simulink model "BEV_Thermal_Management"  (R2025a)
settings: Solver=ode23t  StartTime=0  StopTime=765  MaxStep=5  RelTol=1e-3  AbsTol=1e-3
model workspace: external: MATLAB File BEV_Thermal_Management_param.m (data not in the file)
undefined symbols (not defined in the file): Battery, bulb, cabin_doors_conductivity, cabin_duct_area, cabin_glass_conductivity, cabin_roof_conductivity, cabin_T_init, chiller_area_primary, chiller_N_baffles, chiller_N_tubes, chiller_tube_D, chiller_tube_L, chiller_wall_conductivity, chiller_wall_thickness, compressor_rpm_LUT, condenser_air_area_flow, condenser_air_area_primary, condenser_W, condenser_wall_conductivity, condenser_wall_thickness, coolant_channel_D, coolant_pipe_area, coolant_pipe_D, coolant_T_init, coolant_tank_area, coolant_tank_volume, coolant_valve_D_ratio_max, coolant_valve_D_ratio_min, coolant_valve_displacement, coolant_valve_S_max, cycle, DCDC, Edrive, evaporator_air_area_flow, evaporator_air_area_primary, evaporator_W, evaporator_wall_conductivity, evaporator_wall_thickness, heater_max_power, ModuleType1, outlet, ptc_max_power, pump_speed_max, radiationReflectionShields, radiator_air_area_flow, radiator_air_area_primary, radiator_W, radiator_wall_conductivity, radiator_wall_thickness, refrigerant_alpha_init, refrigerant_pipe_D, transRatio
libraries: fl_lib x264, nesl_utility x91, SimscapeFluids_lib x22, sdl_lib x13, ee_lib x9, nesl_utility_internal x4, slpidlib x3, BatteryProtection x3, batt_lib x2, BatteryCurrentManagement x1, autolibsharedcommon x1, simulink x1
(part 5 of 9)

== system BEV_Thermal_Management/Parallel-Serial Mode Valve ==
  note: Parallel mode flow path: A-D and C-B
      |
      | Serial mode flow path: A-B and C-D
  4-Way Valve : SimscapeFluids_lib/Thermal Liquid/Valves & Orifices/Directional Control Valves/4-Way 3-Position Directional Valve (TL)  open_orifices_pos=fluids.thermal_liquid.valves.directional_control_valves.enum.OpenOrifices4WayPosNeg.PA_BT  open_orifices_neu=fluids.thermal_liquid.valves.directional_control_valves.enum.OpenOrifices4WayNeu.all_closed  open_orifices_neg=fluids.thermal_liquid.valves.directional_control_valves.enum.OpenOrifices4WayPosNeg.PB_AT  neutral_assert_action=simscape.enum.assert.action.none  area_spec=fluids.thermal_liquid.valves.directional_control_valves.enum.area_spec.identical  valve_spec=fluids.thermal_liquid.valves.enum.orifice_spec.linear  del_S_max=coolant_valve_displacement m  area_max=pi * (coolant_valve_D_ratio_max*coolant_pipe_D)^2 / 4 m^2  del_S_TLU=[0 0.002 0.004 0.007 0.017] m  valve_area_TLU=[1e-09, 2.0352e-07, 4.0736e-05, .00011438, .00034356] m^2  del_S_flow_TLU=[0 0.002 0.004 0.007 0.017] m  p_diff_TLU=[-.1, .3, .5, .7] MPa  vol_flow_TLU=[-1e-08, 2.2e-08, 2.8e-08, 3.4e-08; -9e-06, .00015, .0002, .00024; -.00036, .00063, .00081, .00096; -.00054, .00094, .0012, .0014; -.00091, .0016, .002, .0024] m^3/s  mdot_TLU=[-1e-05, 1.7e-05, 2e-05, 2.6e-05; -.002, .0035, .0045, .0053; -.4, .7, .9, 1.06; -1.13, 1.96, 2.5, 3; -3.45, 6, 7.7, 9.13] kg/s  p_diff_TLU_const=[-.1, .3, .5, .7] MPa  vol_flow_TLU_const=[-.0009, .0016, .002, .0024] m^3/s  mdot_TLU_const=[-.9, 1.6, 2, 2.4] kg/s  area_const=1e-4 m^2  T_ref_in=293.15 K  p_ref_in=0.101325 MPa  area_leak=pi * (coolant_valve_D_ratio_min*coolant_pipe_D)^2 / 4 m^2  area=coolant_pipe_area m^2  Cd=0.7  Re_c=12  smoothing_factor=0.01  pressure_recovery=simscape.enum.onoff.on  S_max_PA=coolant_valve_S_max m  del_S_max_PA=coolant_valve_displacement-(coolant_valve_displacement)*(pi * (coolant_valve_D_ratio_min*coolant_pipe_D)^2 / 4)/(pi * (coolant_valve_D_ratio_max*coolant_pipe_D)^2 / 4) m  area_max_PA=pi * (coolant_valve_D_ratio_max*coolant_pipe_D)^2 / 4 m^2  del_S_TLU_PA=[0 0.002 0.004 0.007 0.017] m  valve_area_TLU_PA=[1e-09, 2.0352e-07, 4.0736e-05, .00011438, .00034356] m^2  del_S_flow_TLU_PA=[0 0.002 0.004 0.007 0.017] m  p_diff_TLU_PA=[-.1, .3, .5, .7] MPa  vol_flow_TLU_PA=[-1e-08, 2.2e-08, 2.8e-08, 3.4e-08; -9e-06, .00015, .0002, .00024; -.00036, .00063, .00081, .00096; -.00054, .00094, .0012, .0014; -.00091, .0016, .002, .0024] m^3/s  mdot_TLU_PA=[-1e-05, 1.7e-05, 2e-05, 2.6e-05; -.002, .0035, .0045, .0053; -.4, .7, .9, 1.06; -1.13, 1.96, 2.5, 3; -3.45, 6, 7.7, 9.13] kg/s  area_const_PA=1e-4 m^2  p_diff_TLU_const_PA=[-.1, .3, .5, .7] MPa  vol_flow_TLU_const_PA=[-.0009, .0016, .002, .0024] m^3/s  mdot_TLU_const_PA=[-.9, 1.6, 2, 2.4] kg/s  S_max_PB=-coolant_valve_S_max m  del_S_max_PB=coolant_valve_displacement-(coolant_valve_displacement)*(pi * (coolant_valve_D_ratio_min*coolant_pipe_D)^2 / 4)/(pi * (coolant_valve_D_ratio_max*coolant_pipe_D)^2 / 4) m  area_max_PB=pi * (coolant_valve_D_ratio_max*coolant_pipe_D)^2 / 4 m^2  del_S_TLU_PB=[0 0.002 0.004 0.007 0.017] m  valve_area_TLU_PB=[1e-09, 2.0352e-07, 4.0736e-05, .00011438, .00034356] m^2  del_S_flow_TLU_PB=[0 0.002 0.004 0.007 0.017] m  p_diff_TLU_PB=[-.1, .3, .5, .7] MPa  vol_flow_TLU_PB=[-1e-08, 2.2e-08, 2.8e-08, 3.4e-08; -9e-06, .00015, .0002, .00024; -.00036, .00063, .00081, .00096; -.00054, .00094, .0012, .0014; -.00091, .0016, .002, .0024] m^3/s  mdot_TLU_PB=[-1e-05, 1.7e-05, 2e-05, 2.6e-05; -.002, .0035, .0045, .0053; -.4, .7, .9, 1.06; -1.13, 1.96, 2.5, 3; -3.45, 6, 7.7, 9.13] kg/s  area_const_PB=1e-4 m^2  p_diff_TLU_const_PB=[-.1, .3, .5, .7] MPa  vol_flow_TLU_const_PB=[-.0009, .0016, .002, .0024] m^3/s  mdot_TLU_const_PB=[-.9, 1.6, 2, 2.4] kg/s  S_max_AB=7.5e-3 m  del_S_max_AB=0.005 m  area_max_AB=1e-4 m^2  del_S_TLU_AB=[0, .00125, .0025, .00375, .005] m  valve_area_TLU_AB=[1e-10, 1e-05, 4e-05, 6e-05, .0001] m^2  del_S_flow_TLU_AB=[0, .00125, .0025, .00375, .005] m  p_diff_TLU_AB=[-.1, .3, .5, .7] MPa  vol_flow_TLU_AB=[-1e-08, 2.2e-08, 2.8e-08, 3.4e-08; -9e-06, .00015, .0002, .00024; -.00036, .00063, .00081, .00096; -.00054, .00094, .0012, .0014; -.00091, .0016, .002, .0024] m^3/s  mdot_TLU_AB=[1.7e-05, 2e-05, 2.6e-05; .0035, .0045, .0053; .7, .9, 1.06; 1.96, 2.5, 3; 6, 7.7, 9.13] kg/s  area_const_AB=1e-4 m^2  p_diff_TLU_const_AB=[-.1, .3, .5, .7] MPa  vol_flow_TLU_const_AB=[-.0009, .0016, .002, .0024] m^3/s  mdot_TLU_const_AB=[-.9, 1.6, 2, 2.4] kg/s  S_max_AT=-coolant_valve_S_max m  del_S_max_AT=coolant_valve_displacement-(coolant_valve_displacement)*(pi * (coolant_valve_D_ratio_min*coolant_pipe_D)^2 / 4)/(pi * (coolant_valve_D_ratio_max*coolant_pipe_D)^2 / 4) m  area_max_AT=pi * (coolant_valve_D_ratio_max*coolant_pipe_D)^2 / 4 m^2  del_S_TLU_AT=[0 0.002 0.004 0.007 0.017] m  valve_area_TLU_AT=[1e-09, 2.0352e-07, 4.0736e-05, .00011438, .00034356] m^2  del_S_flow_TLU_AT=[0 0.002 0.004 0.007 0.017] m  p_diff_TLU_AT=[-.1, .3, .5, .7] MPa  vol_flow_TLU_AT=[-1e-08, 2.2e-08, 2.8e-08, 3.4e-08; -9e-06, .00015, .0002, .00024; -.00036, .00063, .00081, .00096; -.00054, .00094, .0012, .0014; -.00091, .0016, .002, .0024] m^3/s  mdot_TLU_AT=[-1e-05, 1.7e-05, 2e-05, 2.6e-05; -.002, .0035, .0045, .0053; -.4, .7, .9, 1.06; -1.13, 1.96, 2.5, 3; -3.45, 6, 7.7, 9.13] kg/s  area_const_AT=1e-4 m^2  p_diff_TLU_const_AT=[-.1, .3, .5, .7] MPa  vol_flow_TLU_const_AT=[-.0009, .0016, .002, .0024] m^3/s  mdot_TLU_const_AT=[-.9, 1.6, 2, 2.4] kg/s  S_max_BT=coolant_valve_S_max m  del_S_max_BT=coolant_valve_displacement-(coolant_valve_displacement)*(pi * (coolant_valve_D_ratio_min*coolant_pipe_D)^2 / 4)/(pi * (coolant_valve_D_ratio_max*coolant_pipe_D)^2 / 4) m  area_max_BT=pi * (coolant_valve_D_ratio_max*coolant_pipe_D)^2 / 4 m^2  del_S_TLU_BT=[0 0.002 0.004 0.007 0.017] m  valve_area_TLU_BT=[1e-09, 2.0352e-07, 4.0736e-05, .00011438, .00034356] m^2  del_S_flow_TLU_BT=[0 0.002 0.004 0.007 0.017] m  p_diff_TLU_BT=[-.1, .3, .5, .7] MPa  vol_flow_TLU_BT=[-1e-08, 2.2e-08, 2.8e-08, 3.4e-08; -9e-06, .00015, .0002, .00024; -.00036, .00063, .00081, .00096; -.00054, .00094, .0012, .0014; -.00091, .0016, .002, .0024] m^3/s  mdot_TLU_BT=[-1e-05, 1.7e-05, 2e-05, 2.6e-05; -.002, .0035, .0045, .0053; -.4, .7, .9, 1.06; -1.13, 1.96, 2.5, 3; -3.45, 6, 7.7, 9.13] kg/s  area_const_BT=1e-4 m^2  p_diff_TLU_const_BT=[-.1, .3, .5, .7] MPa  vol_flow_TLU_const_BT=[-.0009, .0016, .002, .0024] m^3/s  mdot_TLU_const_BT=[-.9, 1.6, 2, 2.4] kg/s  S_max_PT=0 m  del_S_max_PT=0.005 m  area_max_PT=1e-4 m^2  del_S_TLU_PT=[0, .00125, .0025, .00375, .005] m  valve_area_TLU_PT=[1e-10, 1e-05, 4e-05, 6e-05, .0001] m^2  del_S_flow_TLU_PT=[0, .00125, .0025, .00375, .005] m  p_diff_TLU_PT=[-.1, .3, .5, .7] MPa  vol_flow_TLU_PT=[-1e-08, 2.2e-08, 2.8e-08, 3.4e-08; -9e-06, .00015, .0002, .00024; -.00036, .00063, .00081, .00096; -.00054, .00094, .0012, .0014; -.00091, .0016, .002, .0024] m^3/s  mdot_TLU_PT=[1.7e-05, 2e-05, 2.6e-05; .0035, .0045, .0053; .7, .9, 1.06; 1.96, 2.5, 3; 6, 7.7, 9.13] kg/s
      settings: InternalSimscapePortConfiguration="{\"Bottom\":[],\"Left\":[{\"id\":\"A\",\"label\":\"A\",\"type\":\"foundation.thermal_liquid.thermal_liquid\"},{\"id\":\"B\",\"label\":\"B\",\"type\":\"foundation.thermal_liquid.thermal_liquid\"}],\"Right\":[{\"id\":\"S\",\"label\":\"S\",\"type\":\"input\"},{\"id\":\"P\",\"label\":\"P\",\"type\":\"foundation.thermal_liquid.thermal_liquid\"},{\"id\":\"T\",\"label\":\"T\",\"type\":\"foundation.thermal_liquid.thermal_liquid\"}],\"Top\":[]}"
  Battery Coolant Tank : SimscapeFluids_lib/Thermal Liquid/Tanks & Accumulators/Tank (G-TL)  num_inlet=2  volume_total=coolant_tank_volume l  volume_spec=1  tank_area=coolant_tank_area m^2  level_TLU=[0, 3, 5] m  volume_TLU=[0, 4, 6] m^3  inlet_areas_A1B1=[.01, .01] m^2  inlet_height_A2=0.1 m  inlet_area_A2=0.01 m^2  inlet_heights_A2B2=[0, 0] m  inlet_areas_A2B2=[1 1] * coolant_pipe_area m^2  inlet_heights_A2B2C2=[.1, .1, .1] m  inlet_areas_A2B2C2=[.01, .01, .01] m^2  inlet_heights_A2B2C2D2=0.1 * ones(1, 4) m  inlet_areas_A2B2C2D2=0.01 * ones(1, 4) m^2  inlet_heights_A2B2C2D2E2=0.1 * ones(1, 5) m  inlet_areas_A2B2C2D2E2=0.01 * ones(1, 5) m^2  inlet_heights_A2B2C2D2E2F2=0.1 * ones(1, 6) m  inlet_areas_A2B2C2D2E2F2=0.01 * ones(1, 6) m^2  capacity_check=0  max_liquid_capacity=coolant_tank_volume l  g=0 m/s^2  level_specify=on  level_priority=None  level=5 m  level_nominal_specify=off  level_nominal_value=1  level_nominal_unit=m  volume_liquid_specify=on  volume_liquid_priority=High  volume_liquid=0.25 * coolant_tank_volume l  volume_liquid_nominal_specify=off  volume_liquid_nominal_value=1  volume_liquid_nominal_unit=m^3  mass_liquid_specify=off  mass_liquid_priority=None  mass_liquid=5e+3 kg  mass_liquid_nominal_specify=off  mass_liquid_nominal_value=1  mass_liquid_nominal_unit=kg  T_liquid_specify=on  T_liquid_priority=High  T_liquid=coolant_T_init K  T_liquid_nominal_specify=off  T_liquid_nominal_value=1  T_liquid_nominal_unit=K  p_gas_specify=on  p_gas_priority=High  p_gas=coolant_p_init MPa  p_gas_nominal_specify=off  p_gas_nominal_value=1  p_gas_nominal_unit=MPa  T_gas_specify=on  T_gas_priority=High  T_gas=coolant_T_init K  T_gas_nominal_specify=off  T_gas_nominal_value=1  T_gas_nominal_unit=K  rho_gas_specify=off  rho_gas_priority=None  rho_gas=1.2 kg/m^3  rho_gas_nominal_specify=off  rho_gas_nominal_value=1  rho_gas_nominal_unit=kg/m^3
      settings: InternalSimscapePortConfiguration="{\"Bottom\":[],\"Left\":[{\"id\":\"A1\",\"label\":\"A1\",\"type\":\"foundation.gas.gas\"},{\"id\":\"B1\",\"label\":\"B1\",\"type\":\"foundation.gas.gas\"},{\"id\":\"A2\",\"label\":\"A2\",\"type\":\"foundation.thermal_liquid.thermal_liquid\"},{\"id\":\"B2\",\"label\":\"B2\",\"type\":\"foundation.thermal_liquid.thermal_liquid\"}],\"Right\":[{\"id\":\"H1\",\"label\":\"H1\",\"type\":\"foundation.thermal.thermal\"},{\"id\":\"H2\",\"label\":\"H2\",\"type\":\"foundation.thermal.thermal\"}],\"Top\":[{\"id\":\"V_out\",\"label\":\"V\",\"type\":\"output\"},{\"id\":\"L_out\",\"label\":\"L\",\"type\":\"output\"}]}"
  Battery Coolant Tank Heat Transfer : Subsystem
  Bias : Bias  Bias=-1  SaturateOnIntegerOverflow=off
  Cap (G){,1..3} (4 alike) : fl_lib/Gas/Elements/Cap (G)  p_specify=off  p_priority=None  p=0.101325 MPa  p_nominal_specify=off  p_nominal_value=1  p_nominal_unit=MPa  T_specify=off  T_priority=None  T=293.15 K  T_nominal_specify=off  T_nominal_value=1  T_nominal_unit=K
  Coolant Properties : SimscapeFluids_lib/Thermal Liquid/Utilities/Thermal Liquid Properties (TL)  fluid_list=fluids.thermal_liquid.utilities.enum.thermal_liquid_fluid_list.ethylene_glycol  concentration_param_EG=fluids.thermal_liquid.utilities.enum.thermal_liquid_concentration.volume_fraction  concentration_param_PG=fluids.thermal_liquid.utilities.enum.thermal_liquid_concentration.volume_fraction  c_mass_SW=3.5e-3  c_mass_EG=0.1  c_mass_PG=0.1  c_mass_GL=0.1  c_vol_EG=0.4  c_vol_PG=0.1  beta_const_EG=2.1791 GPa  beta_const_PG=2.1791 GPa  beta_const_GL=2.1791 GPa  p_min_EG=0.01 MPa  p_min_PG=0.01 MPa  p_min_GL=0.01 MPa  p_max_EG=50 MPa  p_max_PG=50 MPa  p_max_GL=50 MPa  p_atm=0.101325 MPa  properties_range_check=simscape.enum.assert.action.error
  Coolant Properties2 : SimscapeFluids_lib/Thermal Liquid/Utilities/Thermal Liquid Properties (TL)  Commented=on  fluid_list=fluids.thermal_liquid.utilities.enum.thermal_liquid_fluid_list.ethylene_glycol  concentration_param_EG=fluids.thermal_liquid.utilities.enum.thermal_liquid_concentration.volume_fraction  concentration_param_PG=fluids.thermal_liquid.utilities.enum.thermal_liquid_concentration.volume_fraction  c_mass_SW=3.5e-3  c_mass_EG=0.1  c_mass_PG=0.1  c_mass_GL=0.1  c_vol_EG=0.5  c_vol_PG=0.1  beta_const_EG=2.1791 GPa  beta_const_PG=2.1791 GPa  beta_const_GL=2.1791 GPa  p_min_EG=0.01 MPa  p_min_PG=0.01 MPa  p_min_GL=0.01 MPa  p_max_EG=50 MPa  p_max_PG=50 MPa  p_max_GL=50 MPa  p_atm=0.101325 MPa  properties_range_check=simscape.enum.assert.action.error
  Gain : Gain  Gain=2
  Max Valve Displacement [m] : Gain  Gain=coolant_valve_displacement
  Motor Coolant Tank : SimscapeFluids_lib/Thermal Liquid/Tanks & Accumulators/Tank (G-TL)  num_inlet=2  volume_total=coolant_tank_volume l  volume_spec=1  tank_area=coolant_tank_area m^2  level_TLU=[0, 3, 5] m  volume_TLU=[0, 4, 6] m^3  inlet_areas_A1B1=[.01, .01] m^2  inlet_height_A2=0.1 m  inlet_area_A2=0.01 m^2  inlet_heights_A2B2=[0, 0] m  inlet_areas_A2B2=[1 1] * coolant_pipe_area m^2  inlet_heights_A2B2C2=[.1, .1, .1] m  inlet_areas_A2B2C2=[.01, .01, .01] m^2  inlet_heights_A2B2C2D2=0.1 * ones(1, 4) m  inlet_areas_A2B2C2D2=0.01 * ones(1, 4) m^2  inlet_heights_A2B2C2D2E2=0.1 * ones(1, 5) m  inlet_areas_A2B2C2D2E2=0.01 * ones(1, 5) m^2  inlet_heights_A2B2C2D2E2F2=0.1 * ones(1, 6) m  inlet_areas_A2B2C2D2E2F2=0.01 * ones(1, 6) m^2  capacity_check=0  max_liquid_capacity=coolant_tank_volume l  g=0 m/s^2  level_specify=on  level_priority=None  level=5 m  level_nominal_specify=off  level_nominal_value=1  level_nominal_unit=m  volume_liquid_specify=on  volume_liquid_priority=High  volume_liquid=0.25 * coolant_tank_volume l  volume_liquid_nominal_specify=off  volume_liquid_nominal_value=1  volume_liquid_nominal_unit=m^3  mass_liquid_specify=off  mass_liquid_priority=None  mass_liquid=5e+3 kg  mass_liquid_nominal_specify=off  mass_liquid_nominal_value=1  mass_liquid_nominal_unit=kg  T_liquid_specify=on  T_liquid_priority=High  T_liquid=coolant_T_init K  T_liquid_nominal_specify=off  T_liquid_nominal_value=1  T_liquid_nominal_unit=K  p_gas_specify=on  p_gas_priority=High  p_gas=coolant_p_init MPa  p_gas_nominal_specify=off  p_gas_nominal_value=1  p_gas_nominal_unit=MPa  T_gas_specify=on  T_gas_priority=High  T_gas=coolant_T_init K  T_gas_nominal_specify=off  T_gas_nominal_value=1  T_gas_nominal_unit=K  rho_gas_specify=off  rho_gas_priority=None  rho_gas=1.2 kg/m^3  rho_gas_nominal_specify=off  rho_gas_nominal_value=1  rho_gas_nominal_unit=kg/m^3
      settings: InternalSimscapePortConfiguration="{\"Bottom\":[],\"Left\":[{\"id\":\"A1\",\"label\":\"A1\",\"type\":\"foundation.gas.gas\"},{\"id\":\"B1\",\"label\":\"B1\",\"type\":\"foundation.gas.gas\"},{\"id\":\"A2\",\"label\":\"A2\",\"type\":\"foundation.thermal_liquid.thermal_liquid\"},{\"id\":\"B2\",\"label\":\"B2\",\"type\":\"foundation.thermal_liquid.thermal_liquid\"}],\"Right\":[{\"id\":\"H1\",\"label\":\"H1\",\"type\":\"foundation.thermal.thermal\"},{\"id\":\"H2\",\"label\":\"H2\",\"type\":\"foundation.thermal.thermal\"}],\"Top\":[{\"id\":\"V_out\",\"label\":\"V\",\"type\":\"output\"},{\"id\":\"L_out\",\"label\":\"L\",\"type\":\"output\"}]}"
  Motor Coolant Tank Heat Transfer : Subsystem
  Simulink-PS Converter : nesl_utility/Simulink-PS Converter  PhysicalDomain=network_engine_domain  SubClassName=ps_input  LeftPortType=input  RightPortType=output  PseudoPeriodic=off  Frequencies=[]  NoiseDistribution=none  NoiseParameters=[]  Unit=m  AffineConversion=off  FilteringAndDerivatives=provide  SimscapeFilterOrder=1  InputFilterTimeConstant=0.001  UdotUserProvided=0
  Transfer Fcn : TransferFcn  Denominator=[1 1]
  D : PMIOPort  Side=Left
  A : PMIOPort  Port=2  Side=Left
  B : PMIOPort  Port=3  Side=Right
  C : PMIOPort  Port=4  Side=Right
  wires:
  [cmd_parallel_serial] -> Transfer Fcn/1
  Gain/1 -> Bias/1
  Bias/1 -> Max Valve Displacement [m]/1
  Max Valve Displacement [m]/1 -> Simulink-PS Converter/1
  Transfer Fcn/1 -> Gain/1
  connections:
  4-Way Valve/RConn3 -- Coolant Properties/RConn1 -- Coolant Properties2/RConn1 -- C/RConn1
  4-Way Valve/RConn1 -- Simulink-PS Converter/RConn1
  4-Way Valve/LConn2 -- Motor Coolant Tank/LConn3
  Cap (G)1/LConn1 -- Motor Coolant Tank/LConn2
  Cap (G)/LConn1 -- Motor Coolant Tank/LConn1
  Motor Coolant Tank Heat Transfer/RConn1 -- Motor Coolant Tank/RConn1
  Motor Coolant Tank Heat Transfer/RConn2 -- Motor Coolant Tank/RConn2
  D/RConn1 -- Motor Coolant Tank/LConn4
  Cap (G)2/LConn1 -- Battery Coolant Tank/LConn1
  Cap (G)3/LConn1 -- Battery Coolant Tank/LConn2
  B/RConn1 -- Battery Coolant Tank/LConn4
  4-Way Valve/LConn1 -- Battery Coolant Tank/LConn3
  Battery Coolant Tank Heat Transfer/LConn1 -- Battery Coolant Tank/RConn1
  Battery Coolant Tank Heat Transfer/LConn2 -- Battery Coolant Tank/RConn2
  4-Way Valve/RConn2 -- A/RConn1

== system BEV_Thermal_Management/Radiator ==
  note: The radiator dissipates the heat to the ambient air. This is achieved by air flowing through the radiator. The airflow depends from the fan placed close to the radiator and the vehicle speed
  Air Intake : fl_lib/Moist Air/Elements/Flow Resistance (MA)  delta_p_nominal=5e-4 MPa  mdot_nominal=1 kg/s  rho_nominal=1.2 kg/m^3  area=cabin_duct_area m^2  laminar_fraction=1e-3
  Environment Air : fl_lib/Moist Air/Elements/Reservoir (MA)  pressure_input=true  pressure_spec=foundation.enum.pressure_spec.atmospheric  reservoir_pressure=0.101325 MPa  temperature_input=true  temperature_spec=foundation.enum.temperature_spec.atmospheric  reservoir_temperature=293.15 K  humidity_input=true  humidity_spec=foundation.enum.HumiditySpec.RelativeHumidity  reservoir_RH=0.5  reservoir_x_w=0.01  reservoir_y_w=0.01  reservoir_HR=0.01  reservoir_Tw=287 K  trace_gas_input=true  trace_gas_spec=foundation.enum.trace_gas_spec.mole_fraction  reservoir_x_g=0.001  reservoir_y_g=0.001  water_droplets_input=false  reservoir_r_d=0  RH_ws=1  area_A=cabin_duct_area m^2  input_error_spec=foundation.enum.input_range_error.warn
      settings: InternalSimscapePortConfiguration="{\"Bottom\":[],\"Left\":[{\"id\":\"A\",\"label\":\"A\",\"type\":\"foundation.moist_air.moist_air\"}],\"Right\":[{\"id\":\"T\",\"label\":\"T\",\"type\":\"input\"},{\"id\":\"P\",\"label\":\"P\",\"type\":\"input\"},{\"id\":\"W\",\"label\":\"W\",\"type\":\"input\"},{\"id\":\"G\",\"label\":\"G\",\"type\":\"input\"}],\"Top\":[]}"
  Moist Air Properties : fl_lib/Moist Air/Utilities/Moist Air Properties (MA)  R_a=287.047 J/kg/K  T_TLU=[-56.55, -50 : 10 : -10, -5 : 1 : 5, 10 : 10 : 350]' degC  h_a_TLU=[342.416126230579; 349.005511058471; 359.063577249119; 369.119948684177; 379.175469465129; 389.230944678417; 394.258910928084; 395.264534937366; 396.27017101329; 397.275819932805; 398.281482472874; 399.287159410541; 400.292851523015; 401.298559587728; 402.304284382408; 403.310026685143; 404.315787274435; 409.34489180313; 419.404921755863; 429.468036401264; 439.535033154839; 449.606720928652; 459.683919949603; 469.767460521911; 479.858181001348; 489.956925196484; 500.064539372946; 510.181869006204; 520.309755403634; 530.449032296018; 540.60052248087; 550.765034584465; 560.943359995745; 571.136270013102; 581.344513234296; 591.568813210327; 601.809866375885; 612.068340261954; 622.344871990218; 632.640067043998; 642.95449830646; 653.288705353699; 663.643193987949; 674.018435994423; 684.414869104228; 694.832897145098; 705.272890361557; 715.735185886199; 726.220088344236; 736.727870574087; 747.258774447567; 757.813011774199] kJ/kg  mu_a_TLU=[14.2568883320012; 14.6140127728333; 15.1517277055779; 15.6806860159119; 16.2012351072083; 16.7137043125028; 16.9670071730589; 17.017438062815; 17.0677930842452; 17.1180725309876; 17.1682766951315; 17.2184058672268; 17.2684603362935; 17.3184403898301; 17.3683463138234; 17.4181783927569; 17.4679369096204; 17.7156358640698; 18.2056751785154; 18.68879035749; 19.1652344664982; 19.6352478927873; 20.099059103658; 20.5568853601578; 21.0089333871663; 21.4554000014051; 21.8964726992323; 22.3323302062775; 22.7631429910631; 23.1890737447833; 23.6102778293792; 24.0269036959922; 24.4390932757886; 24.8469823450548; 25.2507008663546; 25.6503733074314; 26.0461189394339; 26.4380521159325; 26.8262825340948; 27.2109154792923; 27.5920520543128; 27.969789394274; 28.3442208682439; 28.7154362685068; 29.0835219883356; 29.4485611890712; 29.8106339572472; 30.1698174524429; 30.5261860464955; 30.8798114546565; 31.2307628592324; 31.5791070262086] s*uPa  k_a_TLU=[19.8808489374933; 20.4162454629695; 21.2248743590758; 22.0232452890903; 22.8117314495857; 23.5906913619588; 23.9767075412237; 24.053639990175; 24.1304826682191; 24.2072359051629; 24.2839000294007; 24.3604753679152; 24.4369622462801; 24.5133609886625; 24.5896719178249; 24.6658953551279; 24.7420316205333; 25.1214164701832; 25.8738283029331; 26.6180150229276; 27.3542674377332; 28.0828634735341; 28.8040686837224; 29.5181367785657; 30.2253101618423; 30.9258204644224; 31.6198890677835; 32.3077276126633; 32.9895384896798; 33.6655153099498; 34.33584335461; 35.0007000027879; 35.6602551380254; 36.3146715334901; 36.9641052165342; 37.6087058133173; 38.248616874307; 38.8839761815308; 39.5149160384798; 40.1415635435708; 40.7640408480637; 41.3824653993118; 41.9969501701893; 42.6076038755117; 43.2145311762238; 43.8178328720941; 44.4176060836121; 45.013944423749; 45.6069381602018; 46.1966743687041; 46.783237077953; 47.3667074066625] mW/m/K  p_min=1 kPa  p_max=inf MPa  T_min=-56.55 degC  T_max=350 degC  properties_range_check=simscape.enum.assert.action.error  p_atm=0.101325 MPa  T_atm=20 degC  enable_droplets=false  R_w=461.523 J/kg/K  p_ws_TLU=[1.71168953425982e-06; 3.93770601979424e-06; 1.28411717710344e-05; 3.80051394873809e-05; .00010323902900209; .000259873810798063; .000401741022116384; .000437454836117844; .000476040820618202; .000517704666185737; .000562664883741207; .000611212677444345; .000657088049117899; .000705987905898279; .000758082381149132; .000813549384183233; .000872574861129522; .00122818386934022; .0023392147667769; .00424668834054807; .00738442748706953; .0123512704340234; .0199458019246787; .0312006356960619; .0474147199263783; .0701823607447713; .10141797792131; .143375967241115; .198665399739302; .270259606559999; .361500961984849; .476101381081492; .618139196722055; .792053183687694; 1.0026345688121; 1.25501792086105; 1.55467186826983; 1.90739066433297; 2.31928772772542; 2.79679245576864; 3.34665187151016; 3.97593907083533; 4.69207105435535; 5.5028394740883; 6.41645928168037; 7.4416425436169; 8.58770832955728; 9.86474556030261; 11.2838558865497; 12.8575218898034; 14.6001810568052; 16.5291642526045] MPa  h_w_vap_TLU=[2836.88241275372; 2837.81392500514; 2838.63937175807; 2838.7309929628; 2838.06905313927; 2836.62597341095; 2835.60023952573; 2835.37006381376; 2835.13143158077; 2834.88429145066; 2834.62859062897; 2500.93420564316; 2498.55329907119; 2496.17495082036; 2493.79885912205; 2491.42474723191; 2489.05236104642; 2477.20875029194; 2453.54955988604; 2429.83856603313; 2406.00136954922; 2381.97406342174; 2357.69101156389; 2333.08088387814; 2308.06565480412; 2282.56034405021; 2256.47287422313; 2229.70428017508; 2202.14968030993; 2173.69998896199; 2144.24368406447; 2113.66758247452; 2081.85585110571; 2048.68725710494; 2014.03141249899; 1977.7449923284; 1939.66849592886; 1899.62342931686; 1857.40930169838; 1812.79975416601; 1765.53721731251; 1715.32525772152; 1661.81700477787; 1604.59703745016; 1543.1534616334; 1476.83692476464; 1404.80240352424; 1325.92091736114; 1238.61667822208; 1140.5102987018; 1027.62017777647; 892.733785613825] kJ/kg  h_w_TLU=[2396.55944251649; 2408.68643343608; 2427.1988031141; 2445.702165897; 2464.18429108356; 2482.62529466839; 2491.82135326629; 2493.6580151792; 2495.49372578218; 2497.32843835745; 2499.16210446923; 2500.99462758899; 2502.83092214066; 2504.6665223621; 2506.50140563013; 2508.335548891; 2510.16892865793; 2519.32352241995; 2537.56068088674; 2555.67742615292; 2573.6403223998; 2591.4109179101; 2608.9455037701; 2626.19492016262; 2643.10444358428; 2659.61377634497; 2675.58278696023; 2696.1846256545; 2716.49989553741; 2736.6235210957; 2756.61216047011; 2776.50561773853; 2796.33378922508; 2816.11979583049; 2835.88181423877; 2855.63430574511; 2875.38889327595; 2895.15500577172; 2914.94035964689; 2934.75132290228; 2954.59319330244; 2974.47041285505; 2994.38673458964; 3014.34535328009; 3034.34900867103; 3054.40006755764; 3074.50058946898; 3094.65237953784; 3114.85703128106; 3135.11596137801; 3155.43043805905; 3175.80160435813] kJ/kg  mu_w_TLU=[6.81365662228272; 7.04953750742707; 7.40970098298307; 7.76991278093907; 8.13017290129507; 8.49048134405107; 8.67065368632907; 8.70668960445667; 8.74272600580827; 8.77876289038387; 8.81480025818347; 8.85083810920707; 8.88687644345467; 8.92291526092627; 8.95895456162187; 8.99499434554147; 9.03103461268507; 9.21124319676307; 9.57169660671907; 9.93219833907507; 10.2927483938311; 10.6533467709871; 11.0139934705431; 11.3746884924991; 11.7354318368551; 12.0962235036111; 12.4570634927671; 12.8179518043231; 13.1788884382791; 13.5398733946351; 13.9009066733911; 14.2619882745471; 14.6231181981031; 14.9842964440591; 15.3455230124151; 15.7067979031711; 16.0681211163271; 16.4294926518831; 16.7909125098391; 17.1523806901951; 17.5138971929511; 17.8754620181071; 18.2370751656631; 18.5987366356191; 18.9604464279751; 19.3222045427311; 19.6840109798871; 20.0458657394431; 20.4077688213991; 20.7697202257551; 21.1317199525111; 21.4937680016671] s*uPa  k_w_TLU=[11.46288215976; 11.941997488935; 12.676358586935; 13.414208884935; 14.155548382935; 14.900377080935; 15.274099879935; 15.348949115735; 15.423833243535; 15.498752263335; 15.573706175135; 15.648694978935; 15.723718674735; 15.798777262535; 15.873870742335; 15.948999114135; 16.024162377935; 16.400502076935; 17.155798374935; 17.914583872935; 18.676858570935; 19.442622468935; 20.211875566935; 20.984617864935; 21.760849362935; 22.540570060935; 23.323779958935; 24.110479056935; 24.900667354935; 25.694344852935; 26.491511550935; 27.292167448935; 28.096312546935; 28.903946844935; 29.715070342935; 30.529683040935; 31.347784938935; 32.169376036935; 32.994456334935; 33.823025832935; 34.655084530935; 35.490632428935; 36.329669526935; 37.172195824935; 38.018211322935; 38.867716020935; 39.720709918935; 40.577193016935; 41.437165314935; 42.300626812935; 43.167577510935; 44.038017408935] mW/m/K  D_w=25 mm^2/s  trace_gas_model=foundation.enum.trace_gas_model.track_fraction  R_g=188.923 J/kg/K  h_g_TLU=[439.555216260064; 444.670268200251; 452.538618847003; 460.487124258496; 468.522588768941; 476.649415958793; 480.74798538725; 481.57054318762; 482.394052398751; 483.218514288831; 484.043930029015; 484.870300696555; 485.697627277859; 486.525910671489; 487.355151691079; 488.185351068185; 489.016509455051; 493.186704139431; 501.599194953048; 510.107689961685; 518.711611080182; 527.410026793075; 536.201764778798; 545.085474203452; 554.059675505208; 563.122805485367; 572.27325096919; 581.509373027928; 590.829525105886; 600.232066705818; 609.715373581392; 619.277845178105; 628.917909922924; 638.634028838794; 648.424697859328; 658.288449140109; 668.223851601449; 678.229510889093; 688.304068901113; 698.44620299875; 708.654624994591; 718.928079991818; 729.265345132425; 739.665228299475; 750.126566808087; 760.648226111439; 771.229098541268; 781.868102096908; 792.564179292476; 803.316296068366; 814.123440770426; 824.984623198037] kJ/kg  mu_g_TLU=[10.8921054191698; 11.2215357085649; 11.7233300740382; 12.2234238147811; 12.7215124453467; 13.2173328890673; 13.4643203184773; 13.5136406274989; 13.562934752385; 13.6122025024997; 13.6614436900741; 13.7106581301692; 13.7598456406398; 13.8090060420983; 13.8581391578796; 13.9072448140062; 13.9563228391538; 14.2012926853717; 14.6890687376044; 15.1738428124161; 15.6554929043332; 16.1339159800463; 16.6090257998657; 17.0807510097148; 17.5490334645512; 18.0138267508952; 18.4750948814453; 18.9328111390399; 19.3869570507278; 19.8375214755778; 20.2844997922255; 20.7278931741254; 21.1677079421287; 21.6039549853963; 22.036649242835; 22.4658092382469; 22.8914566632375; 23.3136160026627; 23.7323141980278; 24.1475803447965; 24.5594454200432; 24.9679420372927; 25.3731042257492; 25.774967231431; 26.1735673380029; 26.5689417053362; 26.9611282240413; 27.350165384404; 27.73609215832; 28.118947892972; 28.4987722151178; 28.8756049449796] s*uPa  k_g_TLU=[10.489430678843; 10.9507672150864; 11.666197960308; 12.392559739764; 13.1299519771612; 13.8778409888416; 14.2554325416312; 14.3312274189707; 14.4071122346908; 14.4830860227061; 14.5591478179508; 14.6352966574703; 14.7115315815553; 14.787851634907; 14.8642558678259; 14.9407433374142; 15.0173131087819; 15.401364480906; 16.1751373988038; 16.9558134611595; 17.7432208682398; 18.5366976599676; 19.3360988502003; 20.1412225692689; 20.9517507672929; 21.7672310558863; 22.5871115634685; 23.4107980865695; 24.2377021890869; 25.0672663781241; 25.8989689893876; 26.732318357514; 27.5668446164644; 28.4020933015927; 29.2376215872816; 30.0729965057542; 30.9077942826816; 31.7416001931033; 32.5740086297993; 33.4046232539953; 34.2330571812868; 35.0589331874899; 35.8818839295189; 36.701552179391; 37.5175910702657; 38.3296643536716; 39.1374466671854; 39.9406238119064; 40.7388930391313; 41.5319633456945; 42.3195557774861; 43.1014037407076] mW/m/K  D_g=16 mm^2/s
  Radiator : SimscapeFluids_lib/Heat Exchangers/Thermal Liquid - Moist Air/Heat Exchanger (TL-MA)  flow_arrangement=fluids.heat_exchangers.enum.FlowArrangementTLMA.Cross  cross_flow_arrangement=fluids.heat_exchangers.enum.CrossFlowArrangementTLMA.MixedUnmixed  R_wall=radiator_wall_thickness / radiator_air_area_primary / radiator_wall_conductivity K/W  wall_thermal_mass=false  mass_wall=1 kg  cp_wall=490 J/(K*kg)  area_A1=coolant_pipe_area m^2  area_B1=coolant_pipe_area m^2  area_A2=cabin_duct_area m^2  area_B2=cabin_duct_area m^2  flow_geometry_TL=fluids.heat_exchangers.enum.FlowGeometryTL.InsideTubes  tube_num_TL=radiator_N_tubes  tube_length_TL=radiator_L m  tube_cross_section_TL=fluids.heat_exchangers.enum.TubeCrossSection.Rectangular  tube_diameter_TL=0.1 m  tube_width_TL=radiator_W m  tube_height_TL=radiator_tube_H m  tube_inner_diameter_TL=0.05 m  tube_outer_diameter_TL=0.1 m  tube_flow_area_TL=0.01 m^2  tube_wetted_perimeter_TL=0.4 m  tube_heat_perimeter_TL=0.4 m  tube_pressure_loss_spec_TL=fluids.heat_exchangers.enum.TubePressureLossSpec.Haaland  tube_loss_coeff_TL=10  tube_local_pressure_loss_spec_TL=fluids.heat_exchangers.enum.LocalLossSpec.AggregateLength  tube_length_add_TL=radiator_tube_Leq m  tube_local_loss_coefficient_TL=0.1  tube_roughness_pressure_TL=15e-6 m  tube_Re_lam_pressure_TL=2000  tube_Re_tur_pressure_TL=4000  tube_shape_factor_generic_TL=64  tube_heat_coeff_spec_TL=fluids.heat_exchangers.enum.TubeHeatCoeffSpec.Gneilinski  tube_colburn_coeff_TL=[.023, .8, .33]  tube_roughness_heat_TL=15e-6 m  tube_Re_lam_heat_TL=2000  tube_Re_tur_heat_TL=4000  tube_Nu_lam_generic_TL=3.66  bank_arrangement_TL=fluids.heat_exchangers.enum.BankArrangement.Inline  bank_num_rows_TL=5  bank_tubes_per_row_TL=5  bank_width_TL=1 m  bank_tube_diameter_TL=0.05 m  bank_longitudinal_pitch_TL=0.15 m  bank_transverse_pitch_TL=0.15 m  bank_pressure_loss_spec_TL=fluids.heat_exchangers.enum.BankPressureLossSpec.Martin  bank_euler_TL=10  bank_heat_coeff_spec_TL=fluids.heat_exchangers.enum.BankHeatCoeffSpec.Martin  bank_colburn_coeff_TL=[.27, .63, .36]  generic_flow_area_TL=0.01 m^2  generic_heat_area_TL=2 m^2  generic_volume_TL=0.05 m^3  generic_loss_coeff_TL=10  generic_colburn_coeff_TL=[.023, .8, .33]  fouling_factor_TL=0.1 m^2*K/kW  fin_area_TL=0 m^2  fin_efficiency_TL=0  p_init_TL=coolant_p_init MPa  T_init_TL=coolant_T_init K  flow_geometry_MA=fluids.heat_exchangers.enum.FlowGeometryMA.Generic  tube_num_MA=1  tube_length_MA=5 m  tube_cross_section_MA=fluids.heat_exchangers.enum.TubeCrossSection.Circular  tube_diameter_MA=0.1 m  tube_width_MA=0.1 m  tube_height_MA=0.1 m  tube_inner_diameter_MA=0.05 m  tube_outer_diameter_MA=0.1 m  tube_flow_area_MA=0.01 m^2  tube_wetted_perimeter_MA=0.4 m  tube_heat_perimeter_MA=0.4 m  tube_pressure_loss_spec_MA=fluids.heat_exchangers.enum.TubePressureLossSpec.Haaland  tube_loss_coeff_MA=10  tube_local_pressure_loss_spec_MA=fluids.heat_exchangers.enum.LocalLossSpec.AggregateLength  tube_length_add_MA=0.1 m  tube_local_loss_coefficient_MA=0.1  tube_roughness_pressure_MA=15e-6 m  tube_Re_lam_pressure_MA=2000  tube_Re_tur_pressure_MA=4000  tube_shape_factor_generic_MA=64  tube_heat_coeff_spec_MA=fluids.heat_exchangers.enum.TubeHeatCoeffSpec.Gneilinski  tube_colburn_coeff_MA=[.023, .8, .33]  tube_roughness_heat_MA=15e-6 m  tube_Re_lam_heat_MA=2000  tube_Re_tur_heat_MA=4000  tube_Nu_lam_generic_MA=3.66  bank_arrangement_MA=fluids.heat_exchangers.enum.BankArrangement.Inline  bank_num_rows_MA=5  bank_tubes_per_row_MA=5  bank_width_MA=1 m  bank_tube_diameter_MA=0.05 m  bank_longitudinal_pitch_MA=0.15 m  bank_transverse_pitch_MA=0.15 m  bank_pressure_loss_spec_MA=fluids.heat_exchangers.enum.BankPressureLossSpec.Martin  bank_euler_MA=10  bank_heat_coeff_spec_MA=fluids.heat_exchangers.enum.BankHeatCoeffSpec.Martin  bank_colburn_coeff_MA=[.27, .63, .36]  generic_flow_area_MA=radiator_air_area_flow m^2  generic_heat_area_MA=radiator_air_area_primary m^2  generic_volume_MA=radiator_air_area_flow * radiator_W m^3  generic_loss_coeff_MA=10  generic_colburn_coeff_MA=[0.27, 0.63, 0.36]  fouling_factor_MA=0.1 m^2*K/kW  fin_area_MA=radiator_air_area_fins m^2  fin_efficiency_MA=0.7  p_init_MA=cabin_p_init MPa  T_init_MA=cabin_T_init K  humidity_spec_MA=foundation.enum.HumiditySpec.RelativeHumidity  RH_init_MA=cabin_RH_init  x_w_init_MA=0.01  y_w_init_MA=0.01  HR_init_MA=0.01  Tw_init_MA=287 K  trace_gas_spec_MA=foundation.enum.trace_gas_spec.mole_fraction  x_g_init_MA=0.001  y_g_init_MA=cabin_CO2_init  r_d_init_MA=0  RH_ws_MA=1  time_constant_cond_MA=1e-3 s  time_constant_evap_MA=1e-3 s  fraction_entrained_MA=1
      settings: InternalSimscapePortConfiguration="{\"Bottom\":[],\"Left\":[{\"id\":\"A1\",\"label\":\"A1\",\"type\":\"foundation.thermal_liquid.thermal_liquid\"},{\"id\":\"B1\",\"label\":\"B1\",\"type\":\"foundation.thermal_liquid.thermal_liquid\"}],\"Right\":[{\"id\":\"A2\",\"label\":\"A2\",\"type\":\"foundation.moist_air.moist_air\"},{\"id\":\"B2\",\"label\":\"B2\",\"type\":\"foundation.moist_air.moist_air\"}],\"Top\":[{\"id\":\"W\",\"label\":\"W\",\"type\":\"output\"}]}"
  Ram Pressure : Subsystem
      settings: PortSchema="{\"entries\":[{\"content\":{\"sides\":[{\"content\":{\"connectorIds\":[\"LConn1\"]},\"type\":\"ConnectorPlacement.EquallySpacedRectSide\",\"uuid\":\"75e3029b-49fb-4aa2-a270-5647ec8f7cc2\"},{\"content\":{\"connectorIds\":[\"RConn1\"],\"side\":\"RIGHT\"},\"type\":\"ConnectorPlacement.EquallySpacedRectSide\",\"uuid\":\"a5773782-5ea1-4526-866f-91c4aa99dd69\"},{\"content\":{\"connectorIds\":[\"LConn2\"],\"side\":\"TOP\"},\"type\":\"ConnectorPlacement.EquallySpacedRectSide\",\"uuid\":\"b1426a6c-920c-4fe3-a6f1-49137f31d8b5\"}]},\"type\":\"ConnectorPlacement.EquallySpacedConnector\",\"uuid\":\"8a57436c-822b-4551-8b15-f9c616e1048b\"}],\"packageUris\":[\"http://schema.mathworks.com/mf0/Connector/R2020b\"],\"version\":\"1.0\"}"
  SC1 : Subsystem
      mask Display: disp(get_param(gcb, 'Name'))
  SC2 : Subsystem
      mask Display: disp(get_param(gcb, 'Name'))
  Simulink-PS Converter : nesl_utility/Simulink-PS Converter  PhysicalDomain=network_engine_domain  SubClassName=ps_input  LeftPortType=input  RightPortType=output  PseudoPeriodic=off  Frequencies=[]  NoiseDistribution=none  NoiseParameters=[]  Unit=degC  AffineConversion=on  FilteringAndDerivatives=provide  SimscapeFilterOrder=1  InputFilterTimeConstant=0.001  UdotUserProvided=0
  Simulink-PS Converter1 : nesl_utility/Simulink-PS Converter  PhysicalDomain=network_engine_domain  SubClassName=ps_input  LeftPortType=input  RightPortType=output  PseudoPeriodic=off  Frequencies=[]  NoiseDistribution=none  NoiseParameters=[]  Unit=MPa  AffineConversion=off  FilteringAndDerivatives=provide  SimscapeFilterOrder=1  InputFilterTimeConstant=0.001  UdotUserProvided=0
  Simulink-PS Converter2 : nesl_utility/Simulink-PS Converter  PhysicalDomain=network_engine_domain  SubClassName=ps_input  LeftPortType=input  RightPortType=output  PseudoPeriodic=off  Frequencies=[]  NoiseDistribution=none  NoiseParameters=[]  Unit=1  AffineConversion=off  FilteringAndDerivatives=provide  SimscapeFilterOrder=1  InputFilterTimeConstant=0.001  UdotUserProvided=0
  Simulink-PS Converter3 : nesl_utility/Simulink-PS Converter  PhysicalDomain=network_engine_domain  SubClassName=ps_input  LeftPortType=input  RightPortType=output  PseudoPeriodic=off  Frequencies=[]  NoiseDistribution=none  NoiseParameters=[]  Unit=1  AffineConversion=off  FilteringAndDerivatives=provide  SimscapeFilterOrder=1  InputFilterTimeConstant=0.001  UdotUserProvided=0
  Simulink-PS Converter4 : nesl_utility/Simulink-PS Converter  PhysicalDomain=network_engine_domain  SubClassName=ps_input  LeftPortType=input  RightPortType=output  PseudoPeriodic=off  Frequencies=[]  NoiseDistribution=none  NoiseParameters=[]  Unit=km/hr  AffineConversion=off  FilteringAndDerivatives=provide  SimscapeFilterOrder=1  InputFilterTimeConstant=0.001  UdotUserProvided=0
  Transfer Fcn : TransferFcn  Denominator=[1 1]
  B : PMIOPort  Side=Left
  A : PMIOPort  Port=2  Side=Right
  T : PMIOPort  Port=3  Side=Right
  wires:
  [RH_env] -> Simulink-PS Converter2/1
  [CO2_env] -> Simulink-PS Converter3/1
  [T_env] -> Simulink-PS Converter/1
  [p_env] -> Simulink-PS Converter1/1
  Transfer Fcn/1 -> Simulink-PS Converter4/1
  [vehSpeed] -> Transfer Fcn/1
  connections:
  B/RConn1 -- SC2/LConn1
  Radiator/LConn1 -- SC1/LConn1
  SC1/RConn1 -- A/RConn1
  Radiator/LConn2 -- SC2/RConn1
  Simulink-PS Converter1/RConn1 -- Environment Air/RConn2
  Simulink-PS Converter2/RConn1 -- Environment Air/RConn3
  Simulink-PS Converter3/RConn1 -- Environment Air/RConn4
  Simulink-PS Converter/RConn1 -- Environment Air/RConn1
  T/RConn1 -- Moist Air Properties/RConn1 -- Radiator/RConn1
  Air Intake/RConn1 -- Radiator/RConn2
  Ram Pressure/RConn1 -- Air Intake/LConn1
  Ram Pressure/LConn1 -- Environment Air/LConn1
  Simulink-PS Converter4/RConn1 -- Ram Pressure/LConn2

== system BEV_Thermal_Management/Radiator Bypass Valve ==
  note: In cold weather, the radiator is bypassed so that heat from the powertrain can be used to warm up the batteries. This is controlled by the 3-way valve that either sends coolant to the radiator or bypasses the radiator.
  note: Go to the radiator
  note: Bypass the radiator
  Bias : Bias  Bias=-1  SaturateOnIntegerOverflow=off
  Flow Resistance (TL) : fl_lib/Thermal Liquid/Elements/Flow Resistance (TL)  delta_p_nominal=0.001 MPa  mdot_nominal=0.3 kg/s  area=coolant_pipe_area m^2  laminar_fraction=1e-3
  Gain : Gain  Gain=2
  Max Valve Displacement [m] : Gain  Gain=coolant_valve_displacement
  Radiator Bypass Valve : SimscapeFluids_lib/Thermal Liquid/Valves & Orifices/Directional Control Valves/3-Way Directional Valve (TL)  open_orifices_pos=fluids.thermal_liquid.valves.directional_control_valves.enum.OpenOrifices3Way.PA  open_orifices_neg=fluids.thermal_liquid.valves.directional_control_valves.enum.OpenOrifices3Way.AT  area_spec=fluids.thermal_liquid.valves.directional_control_valves.enum.area_spec.identical  valve_spec=fluids.thermal_liquid.valves.enum.orifice_spec.linear  del_S_max=coolant_valve_displacement m  area_max=pi * (coolant_valve_D_ratio_max*coolant_pipe_D)^2 / 4 m^2  del_S_TLU=[0 0.002 0.004 0.007 0.017] m  valve_area_TLU=[1e-09, 2.0352e-07, 4.0736e-05, .00011438, .00034356] m^2  del_S_flow_TLU=[0 0.002 0.004 0.007 0.017] m  p_diff_TLU=[-.1, .3, .5, .7] MPa  vol_flow_TLU=1e-3 * [1.7e-05, 2e-05, 2.6e-05; .0035, .0045, .0053; .7, .9, 1.06; 1.96, 2.5, 3; 6, 7.7, 9.13] m^3/s  mdot_TLU=[-1e-05, 1.7e-05, 2e-05, 2.6e-05; -.002, .0035, .0045, .0053; -.4, .7, .9, 1.06; -1.13, 1.96, 2.5, 3; -3.45, 6, 7.7, 9.13] kg/s  T_ref_in=293.15 K  p_ref_in=0.101325 MPa  area_leak=pi * (coolant_valve_D_ratio_min*coolant_pipe_D)^2 / 4 m^2  Cd=0.7  Re_c=12  smoothing_factor=0.01  pressure_recovery=simscape.enum.onoff.on  area=coolant_pipe_area m^2  S_max_PA=coolant_valve_S_max m  del_S_max_PA=coolant_valve_displacement-(coolant_valve_displacement)*(pi * (coolant_valve_D_ratio_min*coolant_pipe_D)^2 / 4)/(pi * (coolant_valve_D_ratio_max*coolant_pipe_D)^2 / 4) m  area_max_PA=pi * (coolant_valve_D_ratio_max*coolant_pipe_D)^2 / 4 m^2  del_S_TLU_PA=[0 0.002 0.004 0.007 0.017] m  valve_area_TLU_PA=[1e-09, 2.0352e-07, 4.0736e-05, .00011438, .00034356] m^2  del_S_flow_TLU_PA=[0 0.002 0.004 0.007 0.017] m  p_diff_TLU_PA=[-.1, .3, .5, .7] MPa  vol_flow_TLU_PA=1e-3 * [1.7e-05, 2e-05, 2.6e-05; .0035, .0045, .0053; .7, .9, 1.06; 1.96, 2.5, 3; 6, 7.7, 9.13] m^3/s  mdot_TLU_PA=[-1e-05, 1.7e-05, 2e-05, 2.6e-05; -.002, .0035, .0045, .0053; -.4, .7, .9, 1.06; -1.13, 1.96, 2.5, 3; -3.45, 6, 7.7, 9.13] kg/s  S_max_AT=-coolant_valve_S_max m  del_S_max_AT=coolant_valve_displacement-(coolant_valve_displacement)*(pi * (coolant_valve_D_ratio_min*coolant_pipe_D)^2 / 4)/(pi * (coolant_valve_D_ratio_max*coolant_pipe_D)^2 / 4) m  area_max_AT=pi * (coolant_valve_D_ratio_max*coolant_pipe_D)^2 / 4 m^2  del_S_TLU_AT=[0 0.002 0.004 0.007 0.017] m  valve_area_TLU_AT=[1e-09, 2.0352e-07, 4.0736e-05, .00011438, .00034356] m^2  del_S_flow_TLU_AT=[0 0.002 0.004 0.007 0.017] m  p_diff_TLU_AT=[-.1, .3, .5, .7] MPa  vol_flow_TLU_AT=1e-3 * [1.7e-05, 2e-05, 2.6e-05; .0035, .0045, .0053; .7, .9, 1.06; 1.96, 2.5, 3; 6, 7.7, 9.13] m^3/s  mdot_TLU_AT=[-1e-05, 1.7e-05, 2e-05, 2.6e-05; -.002, .0035, .0045, .0053; -.4, .7, .9, 1.06; -1.13, 1.96, 2.5, 3; -3.45, 6, 7.7, 9.13] kg/s  S_max_PT=2.5e-3 m  del_S_max_PT=0.005 m  area_max_PT=1e-4 m^2  del_S_TLU_PT=[0, .002, .004, .007, .017] m  valve_area_TLU_PT=[1e-09, 2.0352e-07, 4.0736e-05, .00011438, .00034356] m^2  del_S_flow_TLU_PT=[0, .002, .004, .007, .017] m  p_diff_TLU_PT=[.3, .5, .7] MPa  vol_flow_TLU_PT=1e-3 * [1.7e-05, 2e-05, 2.6e-05; .0035, .0045, .0053; .7, .9, 1.06; 1.96, 2.5, 3; 6, 7.7, 9.13] m^3/s  mdot_TLU_PT=[1.7e-05, 2e-05, 2.6e-05; .0035, .0045, .0053; .7, .9, 1.06; 1.96, 2.5, 3; 6, 7.7, 9.13] kg/s
      settings: InternalSimscapePortConfiguration="{\"Bottom\":[],\"Left\":[{\"id\":\"A\",\"label\":\"A\",\"type\":\"foundation.thermal_liquid.thermal_liquid\"}],\"Right\":[{\"id\":\"S\",\"label\":\"S\",\"type\":\"input\"},{\"id\":\"P\",\"label\":\"P\",\"type\":\"foundation.thermal_liquid.thermal_liquid\"},{\"id\":\"T\",\"label\":\"T\",\"type\":\"foundation.thermal_liquid.thermal_liquid\"}],\"Top\":[]}"
  Simulink-PS Converter : nesl_utility/Simulink-PS Converter  PhysicalDomain=network_engine_domain  SubClassName=ps_input  LeftPortType=input  RightPortType=output  PseudoPeriodic=off  Frequencies=[]  NoiseDistribution=none  NoiseParameters=[]  Unit=m  AffineConversion=off  FilteringAndDerivatives=provide  SimscapeFilterOrder=1  InputFilterTimeConstant=0.001  UdotUserProvided=0
  Transfer Fcn : TransferFcn  Denominator=[1 1]
  B : PMIOPort  Side=Left
  C : PMIOPort  Port=2  Side=Left
  A : PMIOPort  Port=3  Side=Right
  wires:
  Max Valve Displacement [m]/1 -> Simulink-PS Converter/1
  Bias/1 -> Max Valve Displacement [m]/1
  Gain/1 -> Bias/1
  [cmd_rad_bypass] -> Transfer Fcn/1
  Transfer Fcn/1 -> Gain/1
  connections:
  Radiator Bypass Valve/LConn1 -- A/RConn1
  Radiator Bypass Valve/RConn3 -- C/RConn1
  Radiator Bypass Valve/RConn1 -- Simulink-PS Converter/RConn1
  B/RConn1 -- Flow Resistance (TL)/RConn1
  Radiator Bypass Valve/RConn2 -- Flow Resistance (TL)/LConn1

== system BEV_Thermal_Management/Scenario ==
  note: Current vehicle speed
  note: Cabin HVAC
  note: Environment
  AC On/Off : Constant
  CO2 Fraction : Constant  Value=4e-4
  Drive Cycle : Subsystem  mask{time=cycle.t, velocity=cycle.v, mode=cycle.mode}
      mask prompts: time "Drive cycle time vector in sec"; velocity "Drive cycle velocity vector in km/h"; mode "Mode (1=charging, 0=dicharging)"
      mask DialogControl Control1 Prompt: Assign the values for the drive cycle here
      mask Display: disp('Drive Cycle');
  Number of Occupants : Constant
  Pressure [MPa] : Constant  Value=0.101325
  Recirculation On/Off : Constant
  Relative Humidity : Constant  Value=0.5
  Sun Radiaton [W] : Constant  Value=600
  Temperature Setpoint [degC] : Constant  Value=25
  Temperature [degC] : Constant  Value=40
  tag scope: CO2_env=global, N_occupant=global, RH_env=global, T_env=global, T_setpoint=global, ac_onoff=global, chargingMode=global, p_env=global, recirc_onoff=global, sun_Radiation=global, vehSpeedRef=global
  wires:
  Temperature Setpoint [degC]/1 -> [T_setpoint]
  Recirculation On/Off/1 -> [recirc_onoff]
  Number of Occupants/1 -> [N_occupant]
  AC On/Off/1 -> [ac_onoff]
  Pressure [MPa]/1 -> [p_env]
  Temperature [degC]/1 -> [T_env]
  CO2 Fraction/1 -> [CO2_env]
  Relative Humidity/1 -> [RH_env]
  [vehSpeed] -> Drive Cycle/1(Vehicle)
  Drive Cycle/1(Reference) -> [vehSpeedRef]
  Sun Radiaton [W]/1 -> [sun_Radiation]
  Drive Cycle/2(Mode) -> [chargingMode]

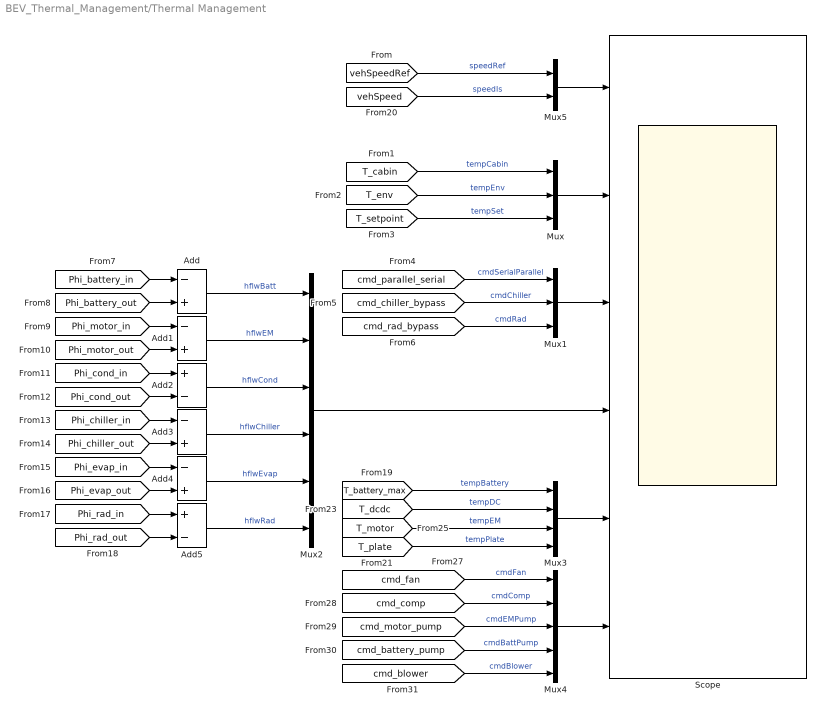
== system BEV_Thermal_Management/Thermal Management ==
  Add{,1,3..4} (4 alike) : Sum  Inputs=-+
  Add2 : Sum  Inputs=+-
  Add5 : Sum  Inputs=+-
  Mux : Mux  Inputs=3
  Mux1 : Mux  Inputs=3
  Mux2 : Mux  Inputs=6
  Mux3 : Mux
  Mux4 : Mux  Inputs=5
  Mux5 : Mux  Inputs=2
  Scope : Scope  NumInputPorts=6
      settings: Title=Vehicle Speed [km/hr]  ActiveDisplayYMinimum=-11.875  ActiveDisplayYMaximum=106.875
  wires:
  Mux4/1 -> Scope/6
  Mux/1 -> Scope/2
  Mux1/1 -> Scope/3
  Mux3/1 -> Scope/5
  Mux5/1 -> Scope/1
  Mux2/1 -> Scope/4
  [T_cabin] -> Mux/1  "tempCabin"
  [vehSpeed] -> Mux5/2  "speedIs"
  [Phi_evap_in] -> Add4/1
  [vehSpeedRef] -> Mux5/1  "speedRef"
  [cmd_fan] -> Mux4/1  "cmdFan"
  [T_battery_max] -> Mux3/1  "tempBattery"
  [cmd_motor_pump] -> Mux4/3  "cmdEMPump"
  Add5/1 -> Mux2/6  "hflwRad"
  [T_motor] -> Mux3/3  "tempEM"
  [cmd_comp] -> Mux4/2  "cmdComp"
  [Phi_motor_out] -> Add1/2
  Add3/1 -> Mux2/4  "hflwChiller"
  [cmd_battery_pump] -> Mux4/4  "cmdBattPump"
  [Phi_rad_in] -> Add5/1
  [Phi_rad_out] -> Add5/2
  Add/1 -> Mux2/1  "hflwBatt"
  [T_env] -> Mux/2  "tempEnv"
  [Phi_battery_in] -> Add/1
  Add2/1 -> Mux2/3  "hflwCond"
  [Phi_cond_out] -> Add2/2
  Add1/1 -> Mux2/2  "hflwEM"
  Add4/1 -> Mux2/5  "hflwEvap"
  [Phi_chiller_out] -> Add3/2
  [Phi_battery_out] -> Add/2
  [T_setpoint] -> Mux/3  "tempSet"
  [T_dcdc] -> Mux3/2  "tempDC"
  [cmd_blower] -> Mux4/5  "cmdBlower"
  [Phi_cond_in] -> Add2/1
  [Phi_motor_in] -> Add1/1
  [cmd_chiller_bypass] -> Mux1/2  "cmdChiller"
  [Phi_chiller_in] -> Add3/1
  [cmd_rad_bypass] -> Mux1/3  "cmdRad"
  [Phi_evap_out] -> Add4/2
  [cmd_parallel_serial] -> Mux1/1  "cmdSerialParallel"
  [T_plate] -> Mux3/4  "tempPlate"

== system BEV_Thermal_Management/Vehicle and Battery ==
  Gain : Gain  Gain=100
  Mux : Mux  Inputs=2
  Scope : Scope  NumInputPorts=4
      settings: TimeSpan=2000  Title=Reference speed vs. Actual speed  ActiveDisplayYMinimum=-16.25  ActiveDisplayYMaximum=146.25  YLabel=Velocity in km/h
  wires:
  Mux/1 -> Scope/1
  [SOCCells] -> Gain/1
  [vehSpeedRef] -> Mux/2
  [vehSpeed] -> Mux/1
  [BatChrgCrnt] -> Scope/2
  Gain/1 -> Scope/3
  [EMTrq] -> Scope/4
